simulink model "rc_radio_channel"  (R2026b)
settings: Solver=VariableStepAuto
undefined symbols (not defined in the file or in its folder): P, Ts
settings Model: Creator=aomar  LastModifiedBy=aomar

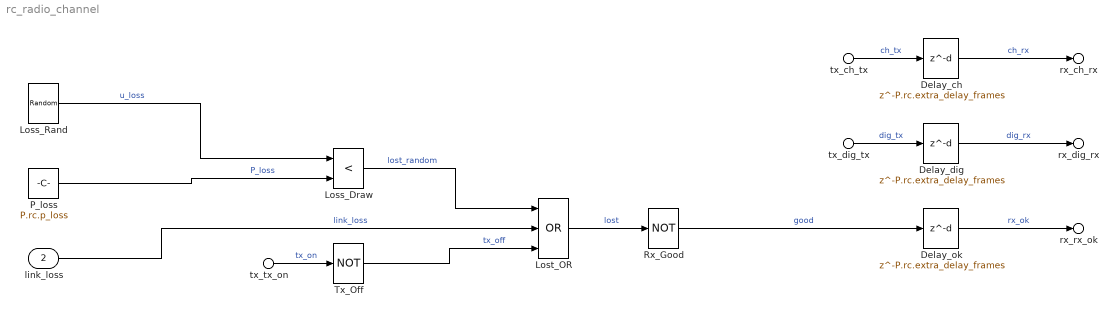
== system rc_radio_channel ==
  tx_tx_on : Inport  PortName=tx  Element=tx_on
  tx_ch_tx : Inport  PortName=tx  Element=ch_tx
  tx_dig_tx : Inport  PortName=tx  Element=dig_tx
  link_loss : Inport  Port=2  OutDataTypeStr=boolean  PortDimensions=1  SampleTime=Ts.rc_frame
  Delay_ch : Delay  DelayLength=P.rc.extra_delay_frames  InitialCondition=P.rc.failsafe_raw
  Delay_dig : Delay  DelayLength=P.rc.extra_delay_frames  InitialCondition=0
  Delay_ok : Delay  DelayLength=P.rc.extra_delay_frames  InitialCondition=0
  Loss_Draw : RelationalOperator  Operator=<  OutDataTypeStr=boolean  RndMeth=Simplest  InputSameDT=off
  Loss_Rand : UniformRandomNumber  Minimum=0  Seed=P.rc.seed  SampleTime=Ts.rc_frame
  Lost_OR : Logic  Operator=OR  Inputs=3  AllPortsSameDT=off  OutDataTypeStr=boolean
  P_loss : Constant  Value=P.rc.p_loss  SampleTime=Ts.rc_frame
  Rx_Good : Logic  Operator=NOT  Inputs=1  AllPortsSameDT=off  OutDataTypeStr=boolean
  Tx_Off : Logic  Operator=NOT  Inputs=1  AllPortsSameDT=off  OutDataTypeStr=boolean
  rx_ch_rx : Outport  PortName=rx  Element=ch_rx
  rx_dig_rx : Outport  PortName=rx  Element=dig_rx
  rx_rx_ok : Outport  PortName=rx  Element=rx_ok
  wires:
  Loss_Rand/1 -> Loss_Draw/1  "u_loss"
  P_loss/1 -> Loss_Draw/2  "P_loss"
  link_loss/1 -> Lost_OR/2  "link_loss"
  tx_tx_on/1 -> Tx_Off/1  "tx_on"
  Loss_Draw/1 -> Lost_OR/1  "lost_random"
  Tx_Off/1 -> Lost_OR/3  "tx_off"
  Lost_OR/1 -> Rx_Good/1  "lost"
  Rx_Good/1 -> Delay_ok/1  "good"
  tx_ch_tx/1 -> Delay_ch/1  "ch_tx"
  tx_dig_tx/1 -> Delay_dig/1  "dig_tx"
  Delay_ch/1 -> rx_ch_rx/1  "ch_rx"
  Delay_dig/1 -> rx_dig_rx/1  "dig_rx"
  Delay_ok/1 -> rx_rx_ok/1  "rx_ok"
